simulink model "Bsw_PMSMCtrl_SimOutput"  (R2025b)
settings: Solver=FixedStepDiscrete  StartTime=0.0  StopTime=0.3  RelTol=1e-3
PreLoadFcn:
  | addpath("Sim\")
  | Sim_PreLoad_PMSMCtrl;
values from neighbouring files (symbols this model uses):
  Par_Cpu_cfCoreFrc = 1.7E+8    [Bsw_PMSMCtrl.sldd]
  Par_Cpu_cfTpwm = 5.0E-5    [Bsw_PMSMCtrl.sldd]
settings Model: DataDictionary=Bsw_PMSMCtrl.sldd  Creator=62555  LastModifiedBy=62555
settings OptimizationCC: DefaultParameterBehavior=Inlined  UseDivisionForNetSlopeComputation=on  DefaultUnderspecifiedDataType=single  EnhancedBackFolding=on  PassReuseOutputArgsAs=Individual arguments  ZeroExternalMemoryAtStartup=off  ZeroInternalMemoryAtStartup=off  OptimizeBlockOrder=speed  DifferentSizesBufferReuse=on  OptimizationCustomize=off  EfficientTunableParamExpr=on
settings DebuggingCC: ParameterTunabilityLossMsg=error
settings SFSimCC: MATLABDynamicMemAlloc=off
settings RTWCC: SystemTargetFile=ert.tlc  GenCodeOnly=on  TemplateMakefile=ert_default_tmf  GenerateReport=on  LaunchReport=on  GPUComputeCapability=3.5  Description=Embedded Coder
settings CodeAppCC: ForceParamTrailComments=on  IgnoreCustomStorageClasses=off  OperatorAnnotations=on  SimulinkDataObjDesc=on  SFDataObjDesc=on  InsertBlockDesc=on
settings ERTTargetCC: ERTCustomFileTemplate=example_file_process.tlc  DynamicArrayContainerType=coder::array  TargetLangStandard=C99 (ISO)  GenerateSampleERTMain=on

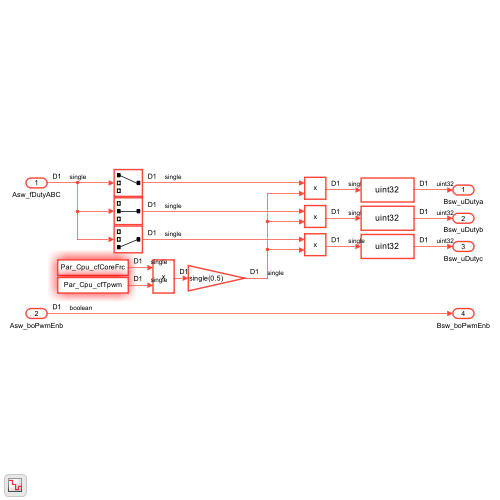
[thumbnail: Simulink's stored preview of the top-level diagram]
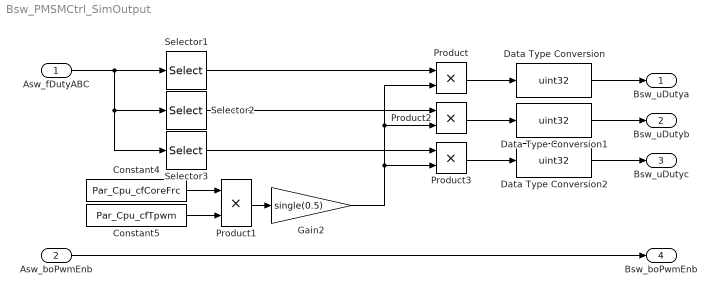
== system Bsw_PMSMCtrl_SimOutput ==
  Asw_fDutyABC : Inport  OutDataTypeStr=single
  Asw_boPwmEnb : Inport  Port=2  OutDataTypeStr=boolean
  Constant4 : Constant  Value=Par_Cpu_cfCoreFrc  OutDataTypeStr=single  SampleTime=-1
  Constant5 : Constant  Value=Par_Cpu_cfTpwm  OutDataTypeStr=single  SampleTime=-1
  Data Type Conversion : DataTypeConversion  OutDataTypeStr=uint32  SaturateOnIntegerOverflow=off  RndMeth=Floor
  Data Type Conversion1 : DataTypeConversion  OutDataTypeStr=uint32  SaturateOnIntegerOverflow=off  RndMeth=Floor
  Data Type Conversion2 : DataTypeConversion  OutDataTypeStr=uint32  SaturateOnIntegerOverflow=off  RndMeth=Floor
  Gain2 : Gain  Gain=single(0.5)
  Product{,1..3} (4 alike) : Product
  Selector1 : Selector  InputPortWidth=3  IndexOptions=Index vector (dialog)  Indices=[1]  OutputSizes=1
  Selector2 : Selector  InputPortWidth=3  IndexOptions=Index vector (dialog)  Indices=[2]  OutputSizes=1
  Selector3 : Selector  InputPortWidth=3  IndexOptions=Index vector (dialog)  Indices=[3]  OutputSizes=1
  Bsw_uDutya : Outport
  Bsw_uDutyb : Outport  Port=2
  Bsw_uDutyc : Outport  Port=3
  Bsw_boPwmEnb : Outport  Port=4
  wires:
  Data Type Conversion1/1 -> Bsw_uDutyb/1
  Product3/1 -> Data Type Conversion2/1
  Gain2/1 -> Product2/2, Product/2, Product3/2
  Data Type Conversion/1 -> Bsw_uDutya/1
  Product1/1 -> Gain2/1
  Asw_fDutyABC/1 -> Selector3/1, Selector2/1, Selector1/1
  Product/1 -> Data Type Conversion/1
  Constant4/1 -> Product1/1
  Product2/1 -> Data Type Conversion1/1
  Constant5/1 -> Product1/2
  Data Type Conversion2/1 -> Bsw_uDutyc/1
  Asw_boPwmEnb/1 -> Bsw_boPwmEnb/1
  Selector2/1 -> Product2/1
  Selector1/1 -> Product/1
  Selector3/1 -> Product3/1
